simulink model "mdl_with_State_Feedback_and_observer"  (R2024b)
settings: Solver=FixedStepAuto  StartTime=0.0  StopTime=Tsim  FixedStep=Ts  RelTol=1e-3
undefined symbols (not defined in the file): input_select, K, k_scale, L, params, plant_ss, q2_f
libraries: SignalEditorBlockLib x1
settings Model: Creator=dsagn  LastModifiedBy=dsagn
settings SolverCC: AlgebraicLoopSolver=TrustRegion
settings DataIOCC: ReturnWorkspaceOutputs=off
settings DebuggingCC: UnconnectedInputMsg=warning  UnconnectedOutputMsg=warning  UnconnectedLineMsg=warning  ArithmeticOperatorsInVariantConditions=warning
settings ModelReferenceCC: EnableRefExpFcnMdlSchedulingChecks=on
settings SFSimCC: CustomCodeUndefinedFunction=UseInterfaceOnly
settings RTWCC: GPUComputeCapability=3.5
settings ConfigComp: CovMetricSettings=de

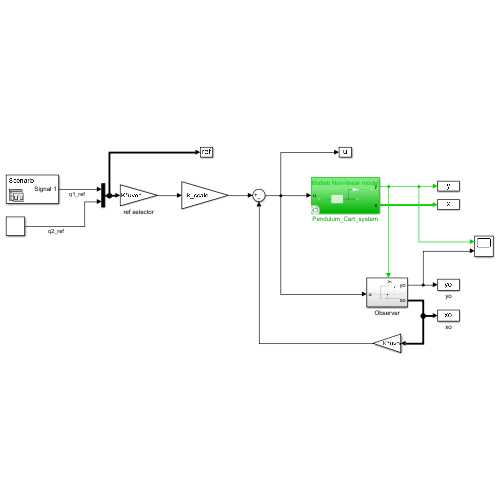
[thumbnail: Simulink's stored preview of the top-level diagram]
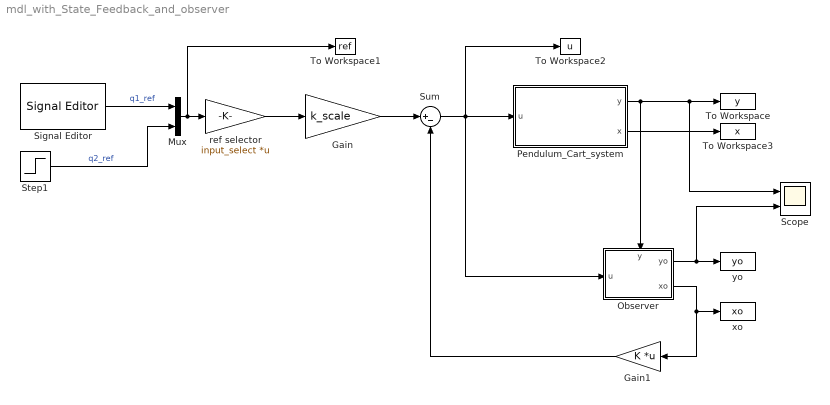
== system mdl_with_State_Feedback_and_observer ==
  Gain : Gain  Gain=k_scale
  Gain1 : Gain  Gain=K  Multiplication=Matrix(K*u) (u vector)
  Mux : Mux  Inputs=2
  Observer : Subsystem  VariantControl=model==1
      settings: PortSchema="{\"entries\":[{\"content\":{\"sides\":[{\"content\":{\"connectorIds\":[\"In1\"]},\"type\":\"ConnectorPlacement.EquallySpacedRectSide\",\"uuid\":\"6f29056e-8395-4acf-a958-2cc2da83c6bb\"},{\"content\":{\"connectorIds\":[\"Out1\",\"Out2\"],\"side\":\"RIGHT\"},\"type\":\"ConnectorPlacement.EquallySpacedRectSide\",\"uuid\":\"2e81148d-cd4e-4b0e-acc4-d8b2ace90135\"},{\"content\":{\"connectorIds\":[\"In2\"],\"side\":\"TOP\"},\"type\":\"ConnectorPlacement.EquallySpacedRectSide\",\"uuid\":\"710f508c-edb8-4863-9098-12d33f6e7baf\"},{\"content\":{\"side\":\"BOTTOM\"},\"type\":\"ConnectorPlacement.EquallySpacedRectSide\",\"uuid\":\"bc3670e7-573f-4e2e-9d5c-9aa118a3e582\"}]},\"type\":\"ConnectorPlacement.EquallySpacedConnector\",\"uuid\":\"432a14f0-84c3-4e6e-8c18-6f5dc974cf86\"}],\"packageUris\":[\"http://schema.mathworks.com/mf0/Connector/R2020b\"],\"version\":\"1.0\"}"
  Pendulum_Cart_system : Subsystem  Variant=on
  Scope : Scope  NumInputPorts=2
  Signal Editor : SignalEditorBlockLib/Signal Editor  FileName=q1_scenario1.mat  ActiveScenario=Scenario  ActiveSignal=Signal 1  IsBus=off  OutputBusObjectStr=Bus: BusObject  SampleTime=0  ZeroCross=off  OutputAfterFinalValue=Setting to zero  Unit=inherit  PreserveSignalName=on  ApplySigPropsToAllScenarios=on  ApplySigPropsToAllSignals=off
  Step1 : Step  After=q2_f  SampleTime=0
  Sum : Sum  Inputs=|+-
  To Workspace : ToWorkspace  VariableName=y  SaveFormat=Timeseries  SampleTime=-1
  To Workspace1 : ToWorkspace  VariableName=ref  SaveFormat=Timeseries  SampleTime=-1
  To Workspace2 : ToWorkspace  VariableName=u  SaveFormat=Timeseries  SampleTime=-1
  To Workspace3 : ToWorkspace  VariableName=x  SaveFormat=Timeseries  SampleTime=-1
  ref selector : Gain  Gain=input_select  Multiplication=Matrix(K*u) (u vector)
  xo : ToWorkspace  VariableName=xo  SaveFormat=Timeseries  SampleTime=-1
  yo : ToWorkspace  VariableName=yo  SaveFormat=Timeseries  SampleTime=-1
  wires:
  ref selector/1 -> Gain/1
  Pendulum_Cart_system/2(x) -> To Workspace3/1
  Pendulum_Cart_system/1(y) -> Scope/1, To Workspace/1, Observer/2(y)
  Step1/1 -> Mux/2  "q2_ref"
  Mux/1 -> To Workspace1/1, ref selector/1
  Signal Editor/1 -> Mux/1  "q1_ref"
  Gain1/1 -> Sum/2
  Gain/1 -> Sum/1
  Sum/1 -> To Workspace2/1, Observer/1(u), Pendulum_Cart_system/1(u)
  Observer/2(xo) -> xo/1, Gain1/1
  Observer/1(yo) -> Scope/2, yo/1

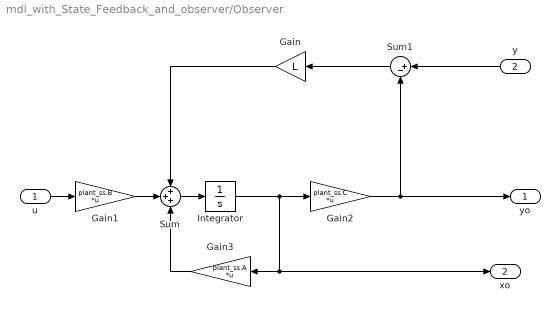
== system mdl_with_State_Feedback_and_observer/Observer ==
  u : Inport
  y : Inport  Port=2
  Gain : Gain  Gain=L
  Gain1 : Gain  Gain=plant_ss.B  Multiplication=Matrix(K*u) (u vector)
  Gain2 : Gain  Gain=plant_ss.C  Multiplication=Matrix(K*u) (u vector)
  Gain3 : Gain  Gain=plant_ss.A  Multiplication=Matrix(K*u) (u vector)
  Integrator : Integrator  InitialCondition=params.IC
  Sum : Sum  Inputs=+++
  Sum1 : Sum  Inputs=|+-
  yo : Outport
  xo : Outport  Port=2
  wires:
  u/1 -> Gain1/1
  Gain1/1 -> Sum/2
  Sum/1 -> Integrator/1
  Gain3/1 -> Sum/3
  Integrator/1 -> Gain2/1, Gain3/1, xo/1
  Gain2/1 -> yo/1, Sum1/2
  Sum1/1 -> Gain/1
  y/1 -> Sum1/1
  Gain/1 -> Sum/1

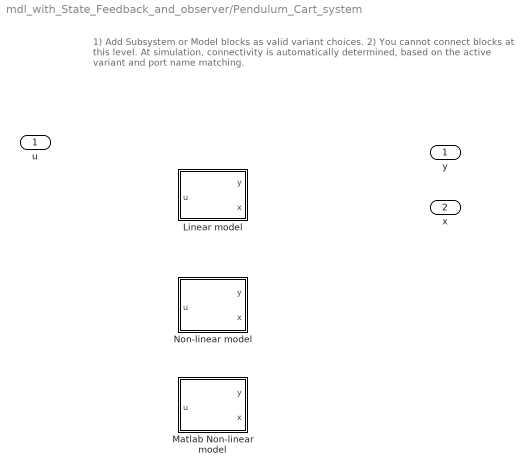
== system mdl_with_State_Feedback_and_observer/Pendulum_Cart_system ==
  note: 1) Add Subsystem or Model blocks as valid variant choices.
      | 2) You cannot connect blocks at this level. At simulation, connectivity is automatically
      | determined, based on the active variant and port name matching.
  u : Inport
  "Linear model " : Subsystem  VariantControl=model==1
  Matlab Non-linear model : Subsystem  VariantControl=model==3
  Non-linear model : Subsystem  VariantControl=model==2
  y : Outport
  x : Outport  Port=2

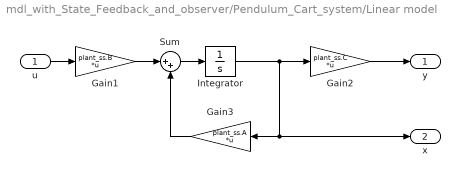
== system mdl_with_State_Feedback_and_observer/Pendulum_Cart_system/Linear model  ==
  u : Inport
  Gain1 : Gain  Gain=plant_ss.B  Multiplication=Matrix(K*u) (u vector)
  Gain2 : Gain  Gain=plant_ss.C  Multiplication=Matrix(K*u) (u vector)
  Gain3 : Gain  Gain=plant_ss.A  Multiplication=Matrix(K*u) (u vector)
  Integrator : Integrator  InitialCondition=params.IC
  Sum : Sum  Inputs=|++
  y : Outport
  x : Outport  Port=2
  wires:
  u/1 -> Gain1/1
  Gain1/1 -> Sum/1
  Sum/1 -> Integrator/1
  Gain3/1 -> Sum/2
  Integrator/1 -> Gain2/1, Gain3/1, x/1
  Gain2/1 -> y/1

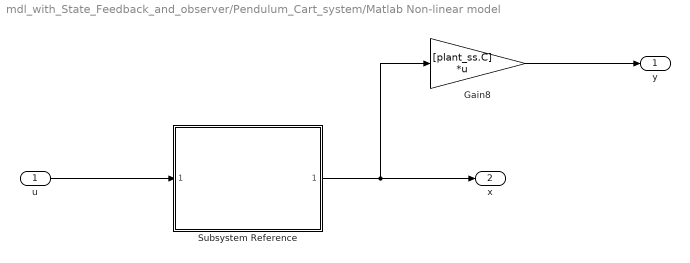
== system mdl_with_State_Feedback_and_observer/Pendulum_Cart_system/Matlab Non-linear model ==
  "u " : Inport
  Gain8 : Gain  Gain=[plant_ss.C]  Multiplication=Matrix(K*u) (u vector)
  Subsystem Reference : Subsystem  ReferencedSubsystem=pendulum_nonlinear_matlab
  y : Outport  VectorParamsAs1DForOutWhenUnconnected=off
  x : Outport  Port=2
  wires:
  Gain8/1 -> y/1
  Subsystem Reference/1 -> Gain8/1, x/1
  "u "/1 -> Subsystem Reference/1

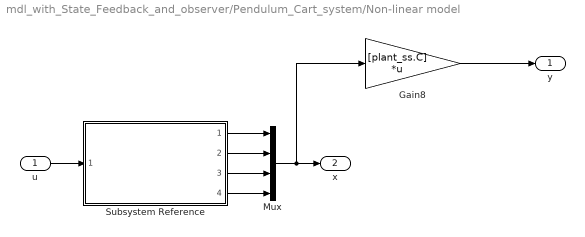
== system mdl_with_State_Feedback_and_observer/Pendulum_Cart_system/Non-linear model ==
  "u " : Inport
  Gain8 : Gain  Gain=[plant_ss.C]  Multiplication=Matrix(K*u) (u vector)
  Mux : Mux
  Subsystem Reference : Subsystem  ReferencedSubsystem=pendulum_nonlinear
  y : Outport  VectorParamsAs1DForOutWhenUnconnected=off
  x : Outport  Port=2
  wires:
  Mux/1 -> Gain8/1, x/1
  Gain8/1 -> y/1
  Subsystem Reference/1 -> Mux/1
  Subsystem Reference/2 -> Mux/2
  Subsystem Reference/3 -> Mux/3
  Subsystem Reference/4 -> Mux/4
  "u "/1 -> Subsystem Reference/1
